simulink model "seondhomework"  (R2024b)
settings: Solver=VariableStepAuto  StartTime=0.0  StopTime=10.0  RelTol=1e-3
values from neighbouring files (symbols this model uses):
  A_orig = [0 1 0 0 ... (first row only)    [secondhomework.m]
  B1st = B_orig(:,1)    [secondhomework.m]
  C_orig = [0 0 1 0]    [secondhomework.m]
  comp = Nu + KT*Nx    [secondhomework.m]
  comp2 = Nu2 + K_orig*Nx2    [secondhomework.m]
  h = 0.20    (= 0.2)    [secondhomework.m]
  initial_output_down_mid = h_mid    (= 0.2)    [secondhomework.m]
  initial_output_up_mid = 0    [secondhomework.m]
  KT = acker(A_orig ,B1st ,desired_poles)    [secondhomework.m]
  Lc = acker(A_orig', C_orig', observer_poles)'    [secondhomework.m]
  slope_mid = tan(angle_mid)    [secondhomework.m]
libraries: simulink x4
settings Model: Creator=moham  LastModifiedBy=moham

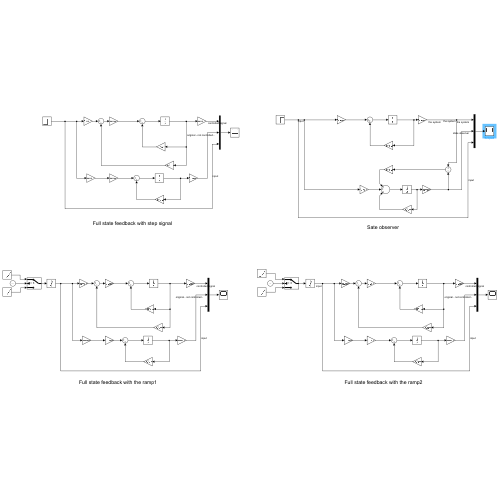
[thumbnail: Simulink's stored preview of the top-level diagram]
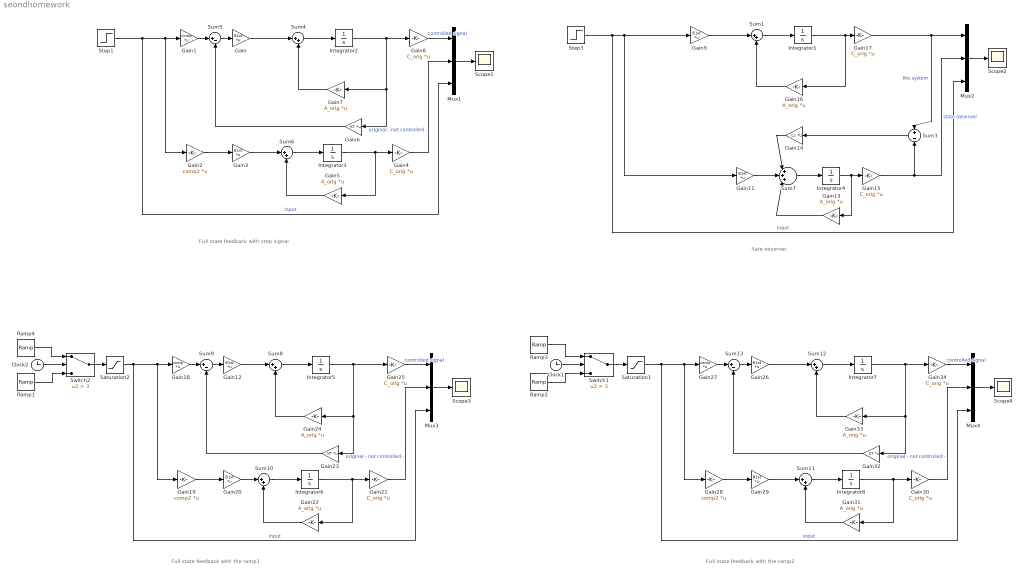
== system seondhomework ==
  note: Full state feedback with step signal
  note: Sate observer
  note: Full state feedback with the ramp1
  note: Full state feedback with the ramp2
  Clock1 : Clock
      settings: Decimation=8
  Clock2 : Clock
      settings: Decimation=8
  Gain{,3,9,11..12,20,26,29} (8 alike) : Gain  Gain=B1st  Multiplication=Matrix(K*u) (u vector)
  Gain1 : Gain  Gain=comp  Multiplication=Matrix(K*u) (u vector)
  Gain{5,7,13,16,22,24,31,33} (8 alike) : Gain  Gain=A_orig  Multiplication=Matrix(K*u) (u vector)
  Gain14 : Gain  Gain=Lc  Multiplication=Matrix(K*u) (u vector)
  Gain{4,8,15,17,21,25,30,34} (8 alike) : Gain  Gain=C_orig  Multiplication=Matrix(K*u) (u vector)
  Gain18 : Gain  Gain=comp  Multiplication=Matrix(K*u) (u vector)
  Gain19 : Gain  Gain=comp2  Multiplication=Matrix(K*u) (u vector)
  Gain2 : Gain  Gain=comp2  Multiplication=Matrix(K*u) (u vector)
  Gain23 : Gain  Gain=KT  Multiplication=Matrix(K*u) (u vector)
  Gain27 : Gain  Gain=comp  Multiplication=Matrix(K*u) (u vector)
  Gain28 : Gain  Gain=comp2  Multiplication=Matrix(K*u) (u vector)
  Gain32 : Gain  Gain=KT  Multiplication=Matrix(K*u) (u vector)
  Gain6 : Gain  Gain=KT  Multiplication=Matrix(K*u) (u vector)
  Integrator{1..8} (8 alike) : Integrator
  Mux{1..4} (4 alike) : Mux  Inputs=3
  Ramp1 : simulink/Sources/Ramp  slope=slope_mid  start=start_time_up_mid  InitialOutput=initial_output_up_mid
  Ramp2 : simulink/Sources/Ramp  slope=tan(angle)  start=1  InitialOutput=0
  Ramp3 : simulink/Sources/Ramp  slope=-tan(angle)  start=3  InitialOutput=h
  Ramp4 : simulink/Sources/Ramp  slope=-slope_mid  start=start_time_down_mid  InitialOutput=initial_output_down_mid
  Saturation1 : Saturate  UpperLimit=h  LowerLimit=0
  Saturation2 : Saturate  UpperLimit=h  LowerLimit=0
  Scope{1..4} (4 alike) : Scope
  Step1 : Step  SampleTime=0
  Step3 : Step  SampleTime=0
  Sum{1,4,6,8,10..12} (7 alike) : Sum  Inputs=|++
  Sum13 : Sum  Inputs=|+-
  Sum3 : Sum  Inputs=+-
  Sum5 : Sum  Inputs=|+-
  Sum7 : Sum  Inputs=|+++|
  Sum9 : Sum  Inputs=|+-
  Switch1 : Switch  Criteria=u2 > Threshold  Threshold=3  SaturateOnIntegerOverflow=off  InputSameDT=off
  Switch2 : Switch  Criteria=u2 > Threshold  Threshold=3  SaturateOnIntegerOverflow=off  InputSameDT=off
  wires:
  Step1/1 -> Gain2/1, Gain1/1, Mux1/3  "input"
  Integrator3/1 -> Gain5/1, Gain4/1
  Gain8/1 -> Mux1/1  "controlled signal"
  Gain2/1 -> Gain3/1
  Gain/1 -> Sum4/1
  Sum4/1 -> Integrator2/1
  Sum6/1 -> Integrator3/1
  Gain4/1 -> Mux1/2  "original - not controlled -"
  Mux1/1 -> Scope1/1
  Gain7/1 -> Sum4/2
  Sum5/1 -> Gain/1
  Gain5/1 -> Sum6/2
  Gain1/1 -> Sum5/1
  Gain3/1 -> Sum6/1
  Gain6/1 -> Sum5/2
  Integrator2/1 -> Gain8/1, Gain7/1, Gain6/1
  Gain16/1 -> Sum1/2
  Mux2/1 -> Scope2/1
  Sum1/1 -> Integrator1/1
  Gain9/1 -> Sum1/1
  Integrator4/1 -> Gain15/1, Gain13/1
  Gain15/1 -> Mux2/2, Sum3/2  "state observer"
  Gain13/1 -> Sum7/3
  Sum7/1 -> Integrator4/1
  Gain11/1 -> Sum7/2
  Gain14/1 -> Sum7/1
  Gain17/1 -> Sum3/1, Mux2/1  "the system"
  Sum3/1 -> Gain14/1
  Step3/1 -> Gain9/1, Gain11/1, Mux2/3  "input"
  Gain19/1 -> Gain20/1
  Gain25/1 -> Mux3/1  "controlled signal"
  Gain22/1 -> Sum10/2
  Gain24/1 -> Sum8/2
  Sum9/1 -> Gain12/1
  Mux3/1 -> Scope3/1
  Gain21/1 -> Mux3/2  "original - not controlled -"
  Sum10/1 -> Integrator6/1
  Sum8/1 -> Integrator5/1
  Integrator5/1 -> Gain25/1, Gain24/1, Gain23/1
  Integrator6/1 -> Gain22/1, Gain21/1
  Saturation2/1 -> Gain19/1, Gain18/1, Mux3/3  "input"
  Gain23/1 -> Sum9/2
  Gain12/1 -> Sum8/1
  Gain18/1 -> Sum9/1
  Gain20/1 -> Sum10/1
  Gain29/1 -> Sum11/1
  Integrator7/1 -> Gain34/1, Gain33/1, Gain32/1
  Integrator8/1 -> Gain31/1, Gain30/1
  Gain27/1 -> Sum13/1
  Gain26/1 -> Sum12/1
  Gain31/1 -> Sum11/2
  Sum12/1 -> Integrator7/1
  Gain34/1 -> Mux4/1  "controlled signal"
  Sum13/1 -> Gain26/1
  Gain28/1 -> Gain29/1
  Mux4/1 -> Scope4/1
  Gain30/1 -> Mux4/2  "original - not controlled -"
  Gain33/1 -> Sum12/2
  Sum11/1 -> Integrator8/1
  Gain32/1 -> Sum13/2
  Ramp4/1 -> Switch2/1
  Clock2/1 -> Switch2/2
  Switch2/1 -> Saturation2/1
  Ramp1/1 -> Switch2/3
  Switch1/1 -> Saturation1/1
  Clock1/1 -> Switch1/2
  Ramp3/1 -> Switch1/1
  Ramp2/1 -> Switch1/3
  Saturation1/1 -> Gain28/1, Gain27/1, Mux4/3  "input"
  Integrator1/1 -> Gain17/1, Gain16/1
